simulink model "nonleaner"  (R2024a)
settings: Solver=VariableStepAuto  StartTime=0.0  StopTime=10  RelTol=1e-3
undefined symbols (not defined in the file): A, B, C, F_mat, G_mat, H_mat, K, K_feedback, K_integral, L, L_red, Nbar
libraries: simulink x5, slpidlib x2
settings Model: Creator=rezax  LastModifiedBy=rezax

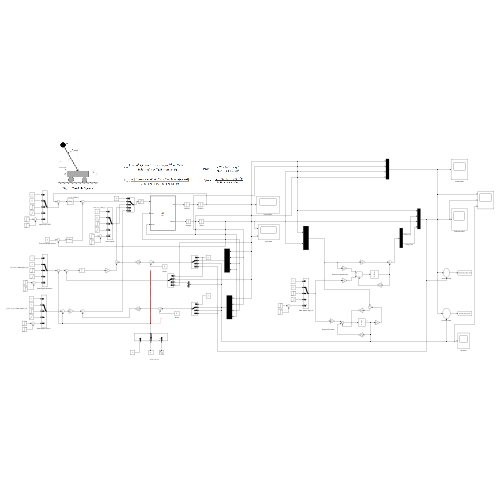
[thumbnail: Simulink's stored preview of the top-level diagram]
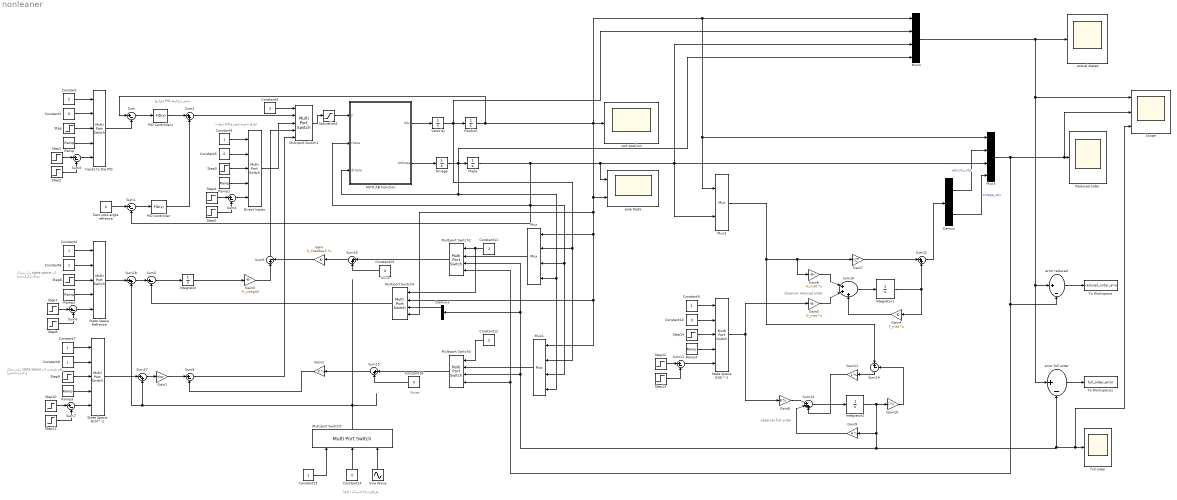
== system nonleaner ==
  note: Noise
  note: ایجاد کننده اغتشاش
  note: observer full order
  note: observer reduced order
  note: کنترلر state space با پیش فاز استاتیکی
  note: کنترلر state space با انتگرال گیر
  note: بدون pid وردوی مستقیم
  note: اولیه PID طراحی شده
  note: Noise
  Constant : Constant  Value=2
  Constant{1,5,10,13..14,16} (6 alike) : Constant  Value=0
  Constant11 : Constant  Value=2
  Constant12 : Constant  Value=2
  Constant{2,4,6..9,15} (7 alike) : Constant
  Constant3 : Constant  Value=3
  Demux : Demux  Outputs=2
  Demux1 : Demux
  Direct Inputs : MultiPortSwitch  Inputs=4  SaturateOnIntegerOverflow=off  InputSameDT=off
  Gain : Gain  Gain=K_feedback  Multiplication=Matrix(K*u)
  Gain1 : Gain  Gain=Nbar
  Gain10 : Gain  Gain=C  Multiplication=Matrix(K*u)
  Gain11 : Gain  Gain=L  Multiplication=Matrix(K*u)
  Gain2 : Gain  Gain=K  Multiplication=Matrix(K*u)
  Gain3 : Gain  Gain=-K_integral
  Gain4 : Gain  Gain=F_mat  Multiplication=Matrix(K*u)
  Gain5 : Gain  Gain=G_mat  Multiplication=Matrix(K*u)
  Gain6 : Gain  Gain=H_mat  Multiplication=Matrix(K*u)
  Gain7 : Gain  Gain=L_red  Multiplication=Matrix(K*u)
  Gain8 : Gain  Gain=B  Multiplication=Matrix(K*u)
  Gain9 : Gain  Gain=A  Multiplication=Matrix(K*u)
  Inputs to the PID : MultiPortSwitch  Inputs=4  SaturateOnIntegerOverflow=off  InputSameDT=off
  Integrator : Integrator
  Integrator1 : Integrator
  Integrator2 : Integrator
  MATLAB Function : MATLAB Function  TreatAsAtomicUnit=on
  Multiport Switch1 : MultiPortSwitch  Inputs=4  SaturateOnIntegerOverflow=off  InputSameDT=off
  Multiport Switch2 : MultiPortSwitch  SaturateOnIntegerOverflow=off  InputSameDT=off
  Multiport Switch3 : MultiPortSwitch  SaturateOnIntegerOverflow=off  InputSameDT=off
  Multiport Switch4 : MultiPortSwitch  SaturateOnIntegerOverflow=off  InputSameDT=off
  Multiport Switch5 : MultiPortSwitch  Inputs=2  SaturateOnIntegerOverflow=off  InputSameDT=off
  Mux{,1,3..4} (4 alike) : Mux
  Mux2 : Mux  Inputs=2
  Omega : Integrator
  PID Controller : slpidlib/PID Controller  Controller=PID  Form=Parallel  TimeDomain=Continuous-time  UseExternalTs=off  SampleTime=-1  IntegratorMethod=Forward Euler  FilterMethod=Forward Euler  ControllerParametersSource=internal  P=-500  I=-1  UseKiTs=off  D=-100  UseExternalDerivativeSource=off  N=100  UseFilter=on  TunerSelectOption=Frequency Response Based  InitialConditionSource=internal  InitialConditionForIntegrator=0  InitialConditionForFilter=0  DifferentiatorICPrevScaledInput=0  ExternalReset=none  TrackingMode=off  Kt=1  LimitOutput=off  SatLimitsSource=internal  UpperSaturationLimit=inf  LowerSaturationLimit=-inf  LinearizeAsGain=on  AntiWindupMode=none  Kb=1  LimitIntegrator=off  UpperIntegratorSaturationLimit=inf  LowerIntegratorSaturationLimit=-inf  POutMin=[]  POutMax=[]  IOutMin=[]  IOutMax=[]  DOutMin=[]  DOutMax=[]  NOutMin=[]  NOutMax=[]  SumOutMin=[]  SumOutMax=[]  SaturationOutMin=[]  SaturationOutMax=[]  PParamMin=[]  PParamMax=[]  IParamMin=[]  IParamMax=[]  DParamMin=[]  DParamMax=[]  NParamMin=[]  NParamMax=[]  KbParamMin=[]  KbParamMax=[]  KtParamMin=[]  KtParamMax=[]  KbOutMin=[]  KbOutMax=[]  KtOutMin=[]  KtOutMax=[]  IntegratorOutMin=[]  IntegratorOutMax=[]  FilterOutMin=[]  FilterOutMax=[]  SumI1OutMin=[]  SumI1OutMax=[]  SumI2OutMin=[]  SumI2OutMax=[]  SumI3OutMin=[]  SumI3OutMax=[]  SumI4OutMin=[]  SumI4OutMax=[]  SumDOutMin=[]  SumDOutMax=[]  DifferentiatorOutMin=[]  DifferentiatorOutMax=[]  FilterDiffOutCoefMin=[]  FilterDiffOutCoefMax=[]  ReciprocalOutMin=[]  ReciprocalOutMax=[]  SumDenOutMin=[]  SumDenOutMax=[]  SumNumOutMin=[]  SumNumOutMax=[]  DivideOutMin=[]  DivideOutMax=[]  UdiffTsProdOutMin=[]  UdiffTsProdOutMax=[]  NTsProdOutMin=[]  NTsProdOutMax=[]  UintegralTsProdOutMin=[]  UintegralTsProdOutMax=[]  UngainTsProdOutMin=[]  UngainTsProdOutMax=[]  ClampingZeroOutDataTypeStr=Inherit: Inherit via back propagation  ClampingZeroOutMin=[]  ClampingZeroOutMax=[]  FilterDenConstantOutDataTypeStr=Inherit: Inherit via back propagation  FilterDenConstantOutMin=[]  FilterDenConstantOutMax=[]  PCopyOutDataTypeStr=Inherit: Inherit via back propagation  PCopyOutMin=[]  PCopyOutMax=[]  NCopyOutDataTypeStr=Inherit: Inherit via back propagation  NCopyOutMin=[]  NCopyOutMax=[]  IntegratorContinuousStateAttributes=''  IntegratorStateMustResolveToSignalObject=off  IntegratorRTWStateStorageClass=Auto  FilterContinuousStateAttributes=''  FilterStateMustResolveToSignalObject=off  FilterRTWStateStorageClass=Auto  ParallelPVariant=InternalParameters  IdealPVariant=Disabled  IVariant=InternalParameters  DVariant=InternalParameters  IntegratorVariant=Continuous  SatVariant=Disabled  AWVariant=Passthrough  PCopyVariant=Disabled  TRVariant=Disabled  FdbkBlocksVariant=Forward  IdealPFdbkVariant=Disabled  SatFdbkVariant=Disabled  DerivativeFilterVariant=ContFilter  NVariant=InternalParameters  NCopyVariant=Disabled  FilterICVariant=InternalICsFilter  IntegratorICVariant=InternalICs  ExternalResetVariant=Disabled  TRSumVariant=Passthrough  SumFdbkVariant=Disabled  SumVariant=Sum_PID  TsampFilterVariant=InternalTs  TsampNgainVariant=Passthrough  TsampIntegralVariant=Disabled_SignalSpec  ExternalSaturationOutDataTypeStr=Inherit: Same as second input  DerivativeSourceVariant=ErrorSignal
  PID Controller1 : slpidlib/PID Controller  Controller=PID  Form=Parallel  TimeDomain=Continuous-time  UseExternalTs=off  SampleTime=-1  IntegratorMethod=Forward Euler  FilterMethod=Forward Euler  ControllerParametersSource=internal  P=40  I=0.8  UseKiTs=off  D=28  UseExternalDerivativeSource=off  N=100  UseFilter=on  TunerSelectOption=Transfer Function Based (PID Tuner App)  InitialConditionSource=internal  InitialConditionForIntegrator=0  InitialConditionForFilter=0  DifferentiatorICPrevScaledInput=0  ExternalReset=none  TrackingMode=off  Kt=1  LimitOutput=off  SatLimitsSource=internal  UpperSaturationLimit=inf  LowerSaturationLimit=-inf  LinearizeAsGain=on  AntiWindupMode=none  Kb=1  LimitIntegrator=off  UpperIntegratorSaturationLimit=inf  LowerIntegratorSaturationLimit=-inf  POutMin=[]  POutMax=[]  IOutMin=[]  IOutMax=[]  DOutMin=[]  DOutMax=[]  NOutMin=[]  NOutMax=[]  SumOutMin=[]  SumOutMax=[]  SaturationOutMin=[]  SaturationOutMax=[]  PParamMin=[]  PParamMax=[]  IParamMin=[]  IParamMax=[]  DParamMin=[]  DParamMax=[]  NParamMin=[]  NParamMax=[]  KbParamMin=[]  KbParamMax=[]  KtParamMin=[]  KtParamMax=[]  KbOutMin=[]  KbOutMax=[]  KtOutMin=[]  KtOutMax=[]  IntegratorOutMin=[]  IntegratorOutMax=[]  FilterOutMin=[]  FilterOutMax=[]  SumI1OutMin=[]  SumI1OutMax=[]  SumI2OutMin=[]  SumI2OutMax=[]  SumI3OutMin=[]  SumI3OutMax=[]  SumI4OutMin=[]  SumI4OutMax=[]  SumDOutMin=[]  SumDOutMax=[]  DifferentiatorOutMin=[]  DifferentiatorOutMax=[]  FilterDiffOutCoefMin=[]  FilterDiffOutCoefMax=[]  ReciprocalOutMin=[]  ReciprocalOutMax=[]  SumDenOutMin=[]  SumDenOutMax=[]  SumNumOutMin=[]  SumNumOutMax=[]  DivideOutMin=[]  DivideOutMax=[]  UdiffTsProdOutMin=[]  UdiffTsProdOutMax=[]  NTsProdOutMin=[]  NTsProdOutMax=[]  UintegralTsProdOutMin=[]  UintegralTsProdOutMax=[]  UngainTsProdOutMin=[]  UngainTsProdOutMax=[]  ClampingZeroOutDataTypeStr=Inherit: Inherit via back propagation  ClampingZeroOutMin=[]  ClampingZeroOutMax=[]  FilterDenConstantOutDataTypeStr=Inherit: Inherit via back propagation  FilterDenConstantOutMin=[]  FilterDenConstantOutMax=[]  PCopyOutDataTypeStr=Inherit: Inherit via back propagation  PCopyOutMin=[]  PCopyOutMax=[]  NCopyOutDataTypeStr=Inherit: Inherit via back propagation  NCopyOutMin=[]  NCopyOutMax=[]  IntegratorContinuousStateAttributes=''  IntegratorStateMustResolveToSignalObject=off  IntegratorRTWStateStorageClass=Auto  FilterContinuousStateAttributes=''  FilterStateMustResolveToSignalObject=off  FilterRTWStateStorageClass=Auto  ParallelPVariant=InternalParameters  IdealPVariant=Disabled  IVariant=InternalParameters  DVariant=InternalParameters  IntegratorVariant=Continuous  SatVariant=Disabled  AWVariant=Passthrough  PCopyVariant=Disabled  TRVariant=Disabled  FdbkBlocksVariant=Forward  IdealPFdbkVariant=Disabled  SatFdbkVariant=Disabled  DerivativeFilterVariant=ContFilter  NVariant=InternalParameters  NCopyVariant=Disabled  FilterICVariant=InternalICsFilter  IntegratorICVariant=InternalICs  ExternalResetVariant=Disabled  TRSumVariant=Passthrough  SumFdbkVariant=Disabled  SumVariant=Sum_PID  TsampFilterVariant=InternalTs  TsampNgainVariant=Passthrough  TsampIntegralVariant=Disabled_SignalSpec  ExternalSaturationOutDataTypeStr=Inherit: Same as second input  DerivativeSourceVariant=ErrorSignal
  Position : Integrator
  Ramp{,1,3..4} (4 alike) : simulink/Sources/Ramp  slope=1  start=0  InitialOutput=0
  Ramp2 : simulink/Sources/Ramp  slope=3  start=0  InitialOutput=0
  Reduced order : Scope
  Saturation1 : Saturate  UpperLimit=50  LowerLimit=-50
  Scope : Scope  NumInputPorts=3
  Sine Wave : Sin  Frequency=2  SampleTime=0
  State Space G(0)^-1 : MultiPortSwitch  Inputs=4  SaturateOnIntegerOverflow=off  InputSameDT=off
  State Space G(0)^-2 : MultiPortSwitch  Inputs=4  SaturateOnIntegerOverflow=off  InputSameDT=off
  State Space Refrence : MultiPortSwitch  Inputs=4  SaturateOnIntegerOverflow=off  InputSameDT=off
  Step{,3,6,9,14} (5 alike) : Step  Time=0  SampleTime=0
  Step{1,4,7,10,12} (5 alike) : Step  SampleTime=0
  Step{2,5,8,11,13} (5 alike) : Step  Time=1.05  SampleTime=0
  Sum{,1,3..9,11,14} (11 alike) : Sum  Inputs=|+-
  Sum10 : Sum  Inputs=|+++
  Sum{2,12,15..18} (6 alike) : Sum  Inputs=|++
  Sum13 : Sum  Inputs=|+++
  Theta : Integrator  InitialCondition=0.05
  To Workspace : ToWorkspace  VariableName=reduced_order_error  SaveFormat=Timeseries  SampleTime=-1
  To Workspace1 : ToWorkspace  VariableName=full_order_error  SaveFormat=Timeseries  SampleTime=-1
  Velocity : Integrator
  Zero pole angle refrence : Constant  Value=0
  actual states : Scope
  cart position : Scope
  error full order : Sum  Inputs=|+-
  error reduced : Sum  Inputs=|+-
  full order : Scope
  pole theta : Scope  NumInputPorts=2
  wires:
  MATLAB Function/2(ddtheta) -> Omega/1
  Omega/1 -> Mux4/4, Theta/1, Mux1/4, Mux/4, MATLAB Function/3(dtheta)
  MATLAB Function/1(ddx) -> Velocity/1
  Velocity/1 -> Mux1/2, Mux/2, Mux4/2, Position/1
  Theta/1 -> Mux3/3, Mux2/2, Mux4/3, pole theta/1, Sum1/2, Mux1/3, Mux/3, MATLAB Function/2(theta)
  Position/1 -> Mux/1, Multiport Switch4/2, Mux1/1, Multiport Switch4/4, pole theta/2, Mux4/1, Mux2/1, Mux3/1, cart position/1, Sum/1
  Sum1/1 -> PID Controller/1
  PID Controller/1 -> Sum2/2
  Sum/1 -> PID Controller1/1
  Sum2/1 -> Multiport Switch1/2
  Constant/1 -> Inputs to the PID/1
  Constant1/1 -> Inputs to the PID/2
  Step/1 -> Inputs to the PID/3
  Ramp/1 -> Inputs to the PID/4
  Step1/1 -> Sum3/1
  Step2/1 -> Sum3/2
  Sum3/1 -> Inputs to the PID/5
  Inputs to the PID/1 -> Sum/2
  Zero pole angle refrence/1 -> Sum1/1
  Constant3/1 -> Multiport Switch1/1
  Ramp1/1 -> Direct Inputs/4
  Step3/1 -> Direct Inputs/3
  Constant4/1 -> Direct Inputs/1
  Constant5/1 -> Direct Inputs/2
  Step4/1 -> Sum4/1
  Sum4/1 -> Direct Inputs/5
  Step5/1 -> Sum4/2
  Direct Inputs/1 -> Multiport Switch1/3
  PID Controller1/1 -> Sum2/1
  Sum5/1 -> Integrator/1
  Multiport Switch1/1 -> Saturation1/1
  Saturation1/1 -> MATLAB Function/1(F)
  State Space Refrence/1 -> Sum18/1
  Step7/1 -> Sum6/1
  Step8/1 -> Sum6/2
  Sum6/1 -> State Space Refrence/5
  Ramp2/1 -> State Space Refrence/4
  Step6/1 -> State Space Refrence/3
  Constant6/1 -> State Space Refrence/2
  Constant2/1 -> State Space Refrence/1
  Ramp3/1 -> State Space G(0)^-1/4
  Constant8/1 -> State Space G(0)^-1/2
  Sum7/1 -> State Space G(0)^-1/5
  Step11/1 -> Sum7/2
  Step9/1 -> State Space G(0)^-1/3
  Step10/1 -> Sum7/1
  Constant7/1 -> State Space G(0)^-1/1
  State Space G(0)^-1/1 -> Sum17/1
  Gain1/1 -> Sum8/1
  Gain2/1 -> Sum8/2
  Sum8/1 -> Multiport Switch1/5
  Integrator/1 -> Gain3/1
  Gain3/1 -> Sum9/1
  Gain/1 -> Sum9/2
  Sum9/1 -> Multiport Switch1/4
  Sum10/1 -> Integrator1/1
  Integrator1/1 -> Gain4/1, Sum12/2
  Gain4/1 -> Sum10/3
  Sum11/1 -> State Space G(0)^-2/5
  Step14/1 -> State Space G(0)^-2/3
  Constant10/1 -> State Space G(0)^-2/2
  Ramp4/1 -> State Space G(0)^-2/4
  Step13/1 -> Sum11/2
  Step12/1 -> Sum11/1
  Constant9/1 -> State Space G(0)^-2/1
  State Space G(0)^-2/1 -> Gain5/1, Gain8/1
  Gain5/1 -> Sum10/2
  Gain6/1 -> Sum10/1
  Mux2/1 -> Gain7/1, Gain6/1, Sum14/1
  Gain7/1 -> Sum12/1
  Sum12/1 -> Demux/1
  Demux/1 -> Mux3/2  "velocity_obs"
  Demux/2 -> Mux3/4  "omega_obs"
  Mux3/1 -> Scope/2, Reduced order/1, Multiport Switch2/4, Multiport Switch3/4, error reduced/2
  Mux4/1 -> error reduced/1, error full order/1, Scope/1, actual states/1
  Integrator2/1 -> Gain9/1, Scope/3, full order/1, error full order/2, Demux1/1, Multiport Switch2/3, Multiport Switch3/3, Gain10/1
  Gain8/1 -> Sum13/1
  Gain9/1 -> Sum13/2
  Gain10/1 -> Sum14/2
  Sum14/1 -> Gain11/1
  Gain11/1 -> Sum13/3
  Sum13/1 -> Integrator2/1
  error reduced/1 -> To Workspace/1
  error full order/1 -> To Workspace1/1
  Mux/1 -> Multiport Switch2/2
  Multiport Switch2/1 -> Sum16/1
  Constant12/1 -> Multiport Switch3/1
  Mux1/1 -> Multiport Switch3/2
  Multiport Switch3/1 -> Sum15/1
  Multiport Switch4/1 -> Sum5/2
  Constant11/1 -> Multiport Switch4/1, Multiport Switch2/1
  Demux1/1 -> Multiport Switch4/3
  Constant15/1 -> Multiport Switch5/1
  Constant14/1 -> Multiport Switch5/2
  Sine Wave/1 -> Multiport Switch5/3
  Multiport Switch5/1 -> Sum18/2, Sum17/2
  Sum15/1 -> Gain2/1
  Sum16/1 -> Gain/1
  Sum17/1 -> Gain1/1
  Sum18/1 -> Sum5/1
  Constant13/1 -> Sum16/2
  Constant16/1 -> Sum15/2

== matlab function nonleaner/MATLAB Function ==
  data: F input; ddx output; theta input; dtheta input; ddtheta output
function [ddx, ddtheta] = fcn(F, theta, dtheta)
% Non-Linear Cart-Pole Dynamics
% Inputs: F (Force), theta (Angle), dtheta (Angular Velocity)

% Parameters
M = 2.0; m = 0.2; l = 0.5; g = 9.81; I = 0.099;

% Trig functions
s = sin(theta);
c = cos(theta);

% Common Denominator
D = (M + m)*(I + m*l^2) - (m*l*c)^2;

% Cart Acceleration (ddx)
num_x = (I + m*l^2)*(F + m*l*dtheta^2*s) - (m*l*c)*(m*g*l*s);
ddx = num_x / D;

% Angular Acceleration (ddtheta)
num_theta = (M + m)*(m*g*l*s) - (m*l*c)*(F + m*l*dtheta^2*s);
ddtheta = num_theta / D;
